simulink model "platform_screen_doors_multibody"  (R2024a)
settings: Solver=ode23t  StartTime=0.0  StopTime=12.5  MaxStep=0.00005  RelTol=1e-4  AbsTol=1e-3  EnableMultiTasking=on
undefined symbols (not defined in the file): X, Y, Z
libraries: fl_lib x27, nesl_utility x13, sm_lib x10, simulink x3, slpidlib x2
settings Model: Creator=USER  LastModifiedBy=Zeus
settings SolverCC: AutoScaleAbsTol=off  AlgebraicLoopSolver=TrustRegion  MaxZcPerStep=1
settings DataIOCC: LimitDataPoints=on  MaxDataPoints=10000  SaveFormat=Array
settings OptimizationCC: ReuseModelBlockBuffer=off  LifeSpan=inf
settings DebuggingCC: UnconnectedInputMsg=warning  UnconnectedOutputMsg=warning  UnconnectedLineMsg=warning  AllowSymbolicDim=off  SubsystemReferenceDiagnosticForUnitTest=warning  SFUnexpectedBacktrackingDiag=warning  SFNoUnconditionalDefaultTransitionDiag=warning  SFExecutionAtInitializationDiag=none  ArithmeticOperatorsInVariantConditions=warning
settings ModelReferenceCC: UpdateModelReferenceTargets=IfOutOfDate  EnableRefExpFcnMdlSchedulingChecks=on
settings SFSimCC: SimUseLocalCustomCode=off  CustomCodeUndefinedFunction=UseInterfaceOnly
settings RTWCC: RTWUseLocalCustomCode=off  GPUComputeCapability=3.5  DLArmComputeVersion=19.05
settings CodeAppCC: StateflowObjectComments=on
settings GRTTargetCC: TargetLangStandard=C89/C90 (ANSI)
settings ConfigComp: CovMetricSettings=dw  CovSaveCumulativeToWorkspaceVar=on  CovSaveSingleToWorkspaceVar=on  CovExternalEMLEnable=off  CovSFcnEnable=off
settings SimscapeCC: SimscapeLogType=all  SimscapeLogDataHistory=10000
settings ExplorerConfigSet: InternalSimMechanicsExplorerSettings=|
  | <ExplorerConfiguration>
  | 
  |   <canonicalview>default</canonicalview>
  | 
  |   <TilePanel>
  |     <TileInfo>
  |       <Tiles Columns="1" Count="1" Height="833" Rows="1" Width="1920">
  |         <Row Weight="1"/>
  |         <Column Weight="1"/>
  |         <Tile Height="1" Width="1" X="0" Y="0"/>
  |       </Tiles>
  |     </TileInfo>
  |     <SceneInfo>
  |       <SceneViewer>
  |         <IsThisViewStd>
  |           <IsStandardView>off</IsStandardView>
  |           <StandardViewName>Front</StandardViewName>
  |         </IsThisViewStd>
  |         <BGColor>
  |           <R>1</R>
  |           <G>1</G>
  |           <B>1</B>
  |           <A>1</A>
  |         </BGColor>
  |         <Camera>
  |           <DoPerspective>off</DoPerspective>
  |           <Position>
  |             <X>0.094040602001582485</X>
  |             <Y>-7.4533549176596825</Y>
  |             <Z>-0.037654221006226174</Z>
  |           </Position>
  |           <Center>
  |             <X>0.094040602001582485</X>
  |             <Y>0</Y>
  |             <Z>-0.037654221006226174</Z>
  |           </Center>
  |           <Up>
  |             <X>0</X>
  |             <Y>0</Y>
  |             <Z>1</Z>
  |           </Up>
  |           <XLim>1.1053593780096338</XLim>
  |           <YLim>1.1053593780096338</YLim>
  |           <ViewLimDist>0.01</ViewLimDist>
  |         </Camera>
  |       </SceneViewer>
  |     </SceneInfo>
  |   </TilePanel>
  | 
  |   <MechEditorPanel>
  |     <GfxPanelCameraMap/>
  |     <Cameras/>
  |     <VideoCreator>
  |       <IncludeTiles>All</IncludeTiles>
  |       <IncludeTime>on</IncludeTime>
  |       <IncludeWorldFrame>off</IncludeWorldFrame>
  |       <PlaybackSpeedRatio>1</PlaybackSpeedRatio>
  |       <FrameRate>30</FrameRate>
  |       <FrameSize>auto</FrameSize>
  |       <VideoFormat>MotionJPEGAVI</VideoFormat>
  |     </VideoCreator>
  |   </MechEditorPanel>
  | 
  |   <PlaybackSettings>
  |     <PlaybackSpeedFactor>1</PlaybackSpeedFactor>
  |   </PlaybackSettings>
  | 
  | </ExplorerConfiguration>

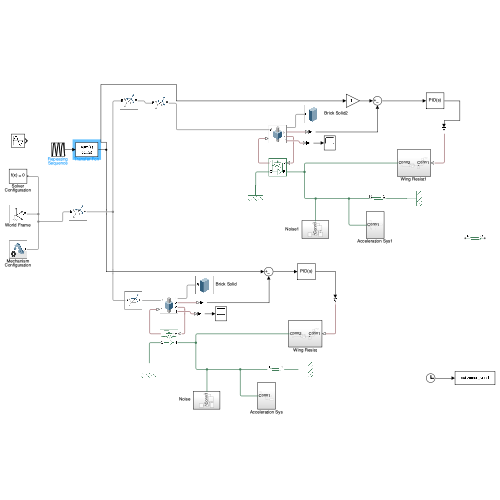
[thumbnail: Simulink's stored preview of the top-level diagram]
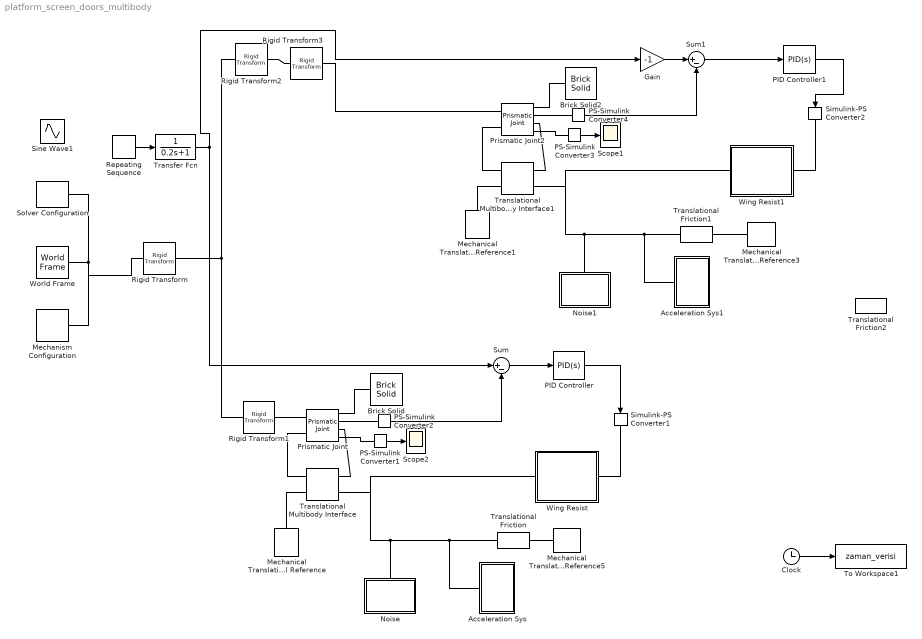
== system platform_screen_doors_multibody ==
  Acceleration Sys : Subsystem
  Acceleration Sys1 : Subsystem
  Brick Solid : sm_lib/Body Elements/Brick Solid  BrickDimensions=[1.9 0.05 0.8]  BrickDimensionsUnits=m  ExportEntireGeometry=off  InertiaType=PointMass  BasedOnType=Density  Density=1000  DensityUnits=kg/m^3  Mass=50  MassUnits=kg  CenterOfMass=[0 0 0]  CenterOfMassUnits=m  MomentsOfInertia=[1 1 1]  MomentsOfInertiaUnits=kg*m^2  ProductsOfInertia=[0 0 0]  ProductsOfInertiaUnits=kg*m^2  GraphicType=FromGeometry  MarkerShape=Sphere  MarkerSize=10  GraphicVisPropType=SimpleVisualProperties  GraphicDiffuseColor=[0.5 0.5 0.5]  GraphicOpacity=1.0  GraphicSpecularColor=[0.5 0.5 0.5 1.0]  GraphicAmbientColor=[0.15 0.15 0.15 1.0]  GraphicEmissiveColor=[0.0 0.0 0.0 1.0]  GraphicShininess=75  DoExposeReferenceFrame=on  SerializedFrames=<Frames/>
  Brick Solid2 : sm_lib/Body Elements/Brick Solid  BrickDimensions=[1.9 0.05 0.8]  BrickDimensionsUnits=m  ExportEntireGeometry=off  InertiaType=PointMass  BasedOnType=Density  Density=1000  DensityUnits=kg/m^3  Mass=50  MassUnits=kg  CenterOfMass=[0 0 0]  CenterOfMassUnits=m  MomentsOfInertia=[1 1 1]  MomentsOfInertiaUnits=kg*m^2  ProductsOfInertia=[0 0 0]  ProductsOfInertiaUnits=kg*m^2  GraphicType=FromGeometry  MarkerShape=Sphere  MarkerSize=10  GraphicVisPropType=SimpleVisualProperties  GraphicDiffuseColor=[0.5 0.5 0.5]  GraphicOpacity=1.0  GraphicSpecularColor=[0.5 0.5 0.5 1.0]  GraphicAmbientColor=[0.15 0.15 0.15 1.0]  GraphicEmissiveColor=[0.0 0.0 0.0 1.0]  GraphicShininess=75  DoExposeReferenceFrame=on  SerializedFrames=<Frames/>
  Clock : Clock
  Gain : Gain  Gain=-1
  Mechanical Translational Reference{,1,3,5} (4 alike) : fl_lib/Mechanical/Translational Elements/Mechanical Translational Reference
  Mechanism Configuration : sm_lib/Utilities/Mechanism Configuration  UniformGravity=Constant  GravityVector=[0 0 0]  GravityVectorUnits=m/s^2  LinearizationDelta=0.001  JointModeTransitionNonlinearIterations=2
  Noise : Subsystem
  Noise1 : Subsystem
  PID Controller : slpidlib/PID Controller  Controller=PID  Form=Parallel  TimeDomain=Continuous-time  UseExternalTs=off  SampleTime=-1  IntegratorMethod=Forward Euler  FilterMethod=Forward Euler  ControllerParametersSource=internal  P=10000  I=4000  UseKiTs=off  D=500  UseExternalDerivativeSource=off  N=100  UseFilter=on  TunerSelectOption=Transfer Function Based (PID Tuner App)  InitialConditionSource=internal  InitialConditionForIntegrator=0  InitialConditionForFilter=0  DifferentiatorICPrevScaledInput=0  ExternalReset=none  TrackingMode=off  Kt=1  LimitOutput=off  SatLimitsSource=internal  UpperSaturationLimit=inf  LowerSaturationLimit=-inf  LinearizeAsGain=on  AntiWindupMode=none  Kb=1  LimitIntegrator=off  UpperIntegratorSaturationLimit=inf  LowerIntegratorSaturationLimit=-inf  POutMin=[]  POutMax=[]  IOutMin=[]  IOutMax=[]  DOutMin=[]  DOutMax=[]  NOutMin=[]  NOutMax=[]  SumOutMin=[]  SumOutMax=[]  SaturationOutMin=[]  SaturationOutMax=[]  PParamMin=[]  PParamMax=[]  IParamMin=[]  IParamMax=[]  DParamMin=[]  DParamMax=[]  NParamMin=[]  NParamMax=[]  KbParamMin=[]  KbParamMax=[]  KtParamMin=[]  KtParamMax=[]  KbOutMin=[]  KbOutMax=[]  KtOutMin=[]  KtOutMax=[]  IntegratorOutMin=[]  IntegratorOutMax=[]  FilterOutMin=[]  FilterOutMax=[]  SumI1OutMin=[]  SumI1OutMax=[]  SumI2OutMin=[]  SumI2OutMax=[]  SumI3OutMin=[]  SumI3OutMax=[]  SumI4OutMin=[]  SumI4OutMax=[]  SumDOutMin=[]  SumDOutMax=[]  DifferentiatorOutMin=[]  DifferentiatorOutMax=[]  FilterDiffOutCoefMin=[]  FilterDiffOutCoefMax=[]  ReciprocalOutMin=[]  ReciprocalOutMax=[]  SumDenOutMin=[]  SumDenOutMax=[]  SumNumOutMin=[]  SumNumOutMax=[]  DivideOutMin=[]  DivideOutMax=[]  UdiffTsProdOutMin=[]  UdiffTsProdOutMax=[]  NTsProdOutMin=[]  NTsProdOutMax=[]  UintegralTsProdOutMin=[]  UintegralTsProdOutMax=[]  UngainTsProdOutMin=[]  UngainTsProdOutMax=[]  ClampingZeroOutDataTypeStr=Inherit: Inherit via back propagation  ClampingZeroOutMin=[]  ClampingZeroOutMax=[]  FilterDenConstantOutDataTypeStr=Inherit: Inherit via back propagation  FilterDenConstantOutMin=[]  FilterDenConstantOutMax=[]  PCopyOutDataTypeStr=Inherit: Inherit via back propagation  PCopyOutMin=[]  PCopyOutMax=[]  NCopyOutDataTypeStr=Inherit: Inherit via back propagation  NCopyOutMin=[]  NCopyOutMax=[]  IntegratorContinuousStateAttributes=''  IntegratorStateMustResolveToSignalObject=off  IntegratorRTWStateStorageClass=Auto  FilterContinuousStateAttributes=''  FilterStateMustResolveToSignalObject=off  FilterRTWStateStorageClass=Auto  ParallelPVariant=InternalParameters  IdealPVariant=Disabled  IVariant=InternalParameters  DVariant=InternalParameters  IntegratorVariant=Continuous  SatVariant=Disabled  AWVariant=Passthrough  PCopyVariant=Disabled  TRVariant=Disabled  FdbkBlocksVariant=Forward  IdealPFdbkVariant=Disabled  SatFdbkVariant=Disabled  DerivativeFilterVariant=ContFilter  NVariant=InternalParameters  NCopyVariant=Disabled  FilterICVariant=InternalICsFilter  IntegratorICVariant=InternalICs  ExternalResetVariant=Disabled  TRSumVariant=Passthrough  SumFdbkVariant=Disabled  SumVariant=Sum_PID  TsampFilterVariant=InternalTs  TsampNgainVariant=Passthrough  TsampIntegralVariant=Disabled_SignalSpec  ExternalSaturationOutDataTypeStr=Inherit: Same as second input  DerivativeSourceVariant=ErrorSignal
  PID Controller1 : slpidlib/PID Controller  Controller=PID  Form=Parallel  TimeDomain=Continuous-time  UseExternalTs=off  SampleTime=-1  IntegratorMethod=Forward Euler  FilterMethod=Forward Euler  ControllerParametersSource=internal  P=10000  I=4000  UseKiTs=off  D=500  UseExternalDerivativeSource=off  N=100  UseFilter=on  TunerSelectOption=Transfer Function Based (PID Tuner App)  InitialConditionSource=internal  InitialConditionForIntegrator=0  InitialConditionForFilter=0  DifferentiatorICPrevScaledInput=0  ExternalReset=none  TrackingMode=off  Kt=1  LimitOutput=off  SatLimitsSource=internal  UpperSaturationLimit=inf  LowerSaturationLimit=-inf  LinearizeAsGain=on  AntiWindupMode=none  Kb=1  LimitIntegrator=off  UpperIntegratorSaturationLimit=inf  LowerIntegratorSaturationLimit=-inf  POutMin=[]  POutMax=[]  IOutMin=[]  IOutMax=[]  DOutMin=[]  DOutMax=[]  NOutMin=[]  NOutMax=[]  SumOutMin=[]  SumOutMax=[]  SaturationOutMin=[]  SaturationOutMax=[]  PParamMin=[]  PParamMax=[]  IParamMin=[]  IParamMax=[]  DParamMin=[]  DParamMax=[]  NParamMin=[]  NParamMax=[]  KbParamMin=[]  KbParamMax=[]  KtParamMin=[]  KtParamMax=[]  KbOutMin=[]  KbOutMax=[]  KtOutMin=[]  KtOutMax=[]  IntegratorOutMin=[]  IntegratorOutMax=[]  FilterOutMin=[]  FilterOutMax=[]  SumI1OutMin=[]  SumI1OutMax=[]  SumI2OutMin=[]  SumI2OutMax=[]  SumI3OutMin=[]  SumI3OutMax=[]  SumI4OutMin=[]  SumI4OutMax=[]  SumDOutMin=[]  SumDOutMax=[]  DifferentiatorOutMin=[]  DifferentiatorOutMax=[]  FilterDiffOutCoefMin=[]  FilterDiffOutCoefMax=[]  ReciprocalOutMin=[]  ReciprocalOutMax=[]  SumDenOutMin=[]  SumDenOutMax=[]  SumNumOutMin=[]  SumNumOutMax=[]  DivideOutMin=[]  DivideOutMax=[]  UdiffTsProdOutMin=[]  UdiffTsProdOutMax=[]  NTsProdOutMin=[]  NTsProdOutMax=[]  UintegralTsProdOutMin=[]  UintegralTsProdOutMax=[]  UngainTsProdOutMin=[]  UngainTsProdOutMax=[]  ClampingZeroOutDataTypeStr=Inherit: Inherit via back propagation  ClampingZeroOutMin=[]  ClampingZeroOutMax=[]  FilterDenConstantOutDataTypeStr=Inherit: Inherit via back propagation  FilterDenConstantOutMin=[]  FilterDenConstantOutMax=[]  PCopyOutDataTypeStr=Inherit: Inherit via back propagation  PCopyOutMin=[]  PCopyOutMax=[]  NCopyOutDataTypeStr=Inherit: Inherit via back propagation  NCopyOutMin=[]  NCopyOutMax=[]  IntegratorContinuousStateAttributes=''  IntegratorStateMustResolveToSignalObject=off  IntegratorRTWStateStorageClass=Auto  FilterContinuousStateAttributes=''  FilterStateMustResolveToSignalObject=off  FilterRTWStateStorageClass=Auto  ParallelPVariant=InternalParameters  IdealPVariant=Disabled  IVariant=InternalParameters  DVariant=InternalParameters  IntegratorVariant=Continuous  SatVariant=Disabled  AWVariant=Passthrough  PCopyVariant=Disabled  TRVariant=Disabled  FdbkBlocksVariant=Forward  IdealPFdbkVariant=Disabled  SatFdbkVariant=Disabled  DerivativeFilterVariant=ContFilter  NVariant=InternalParameters  NCopyVariant=Disabled  FilterICVariant=InternalICsFilter  IntegratorICVariant=InternalICs  ExternalResetVariant=Disabled  TRSumVariant=Passthrough  SumFdbkVariant=Disabled  SumVariant=Sum_PID  TsampFilterVariant=InternalTs  TsampNgainVariant=Passthrough  TsampIntegralVariant=Disabled_SignalSpec  ExternalSaturationOutDataTypeStr=Inherit: Same as second input  DerivativeSourceVariant=ErrorSignal
  PS-Simulink Converter{1..4} (4 alike) : nesl_utility/PS-Simulink Converter  PhysicalDomain=network_engine_domain  SubClassName=ps_output  LeftPortType=input  RightPortType=output  PseudoPeriodic=off  Frequencies=[]  VectorFormat=inherit  Unit=inherit  AffineConversion=off
  Prismatic Joint : sm_lib/Joints/Prismatic Joint  JointMode=Normal  CompositeWrenchDir=FollowerOnBase  CompositeWrenchFrame=BaseFrame  SenseConstraintForce=off  SenseConstraintTorque=off  SenseTotalForce=off  SenseTotalTorque=off  PositionTargetSpecify=off  PositionTargetPriority=High  PositionTargetValue=0  PositionTargetValueUnits=m  VelocityTargetSpecify=off  VelocityTargetPriority=High  VelocityTargetValue=0  VelocityTargetValueUnits=m/s  EquilibriumPosition=0  EquilibriumPositionUnits=m  SpringStiffness=50  SpringStiffnessUnits=N/m  DampingCoefficient=10  DampingCoefficientUnits=N/(m/s)  LowerLimitSpecify=on  LowerLimitBound=0  LowerLimitBoundUnits=m  LowerLimitStiffness=1e6  LowerLimitStiffnessUnits=N/m  LowerLimitDamping=1e3  LowerLimitDampingUnits=N/(m/s)  LowerLimitTransitionRegionWidth=1e-4  LowerLimitTransitionRegionWidthUnits=m  UpperLimitSpecify=on  UpperLimitBound=0.8  UpperLimitBoundUnits=m  UpperLimitStiffness=1e6  UpperLimitStiffnessUnits=N/m  UpperLimitDamping=1e3  UpperLimitDampingUnits=N/(m/s)  UpperLimitTransitionRegionWidth=1e-4  UpperLimitTransitionRegionWidthUnits=m  TorqueActuationMode=InputTorque  MotionActuationMode=ComputedMotion  SensePosition=on  SenseVelocity=on  SenseAcceleration=off  SenseTorqueForce=on  SenseLowerLimitTorqueForce=off  SenseUpperLimitTorqueForce=off
  Prismatic Joint2 : sm_lib/Joints/Prismatic Joint  JointMode=Normal  CompositeWrenchDir=FollowerOnBase  CompositeWrenchFrame=BaseFrame  SenseConstraintForce=off  SenseConstraintTorque=off  SenseTotalForce=off  SenseTotalTorque=off  PositionTargetSpecify=off  PositionTargetPriority=High  PositionTargetValue=0  PositionTargetValueUnits=m  VelocityTargetSpecify=off  VelocityTargetPriority=High  VelocityTargetValue=0  VelocityTargetValueUnits=m/s  EquilibriumPosition=0  EquilibriumPositionUnits=m  SpringStiffness=50  SpringStiffnessUnits=N/m  DampingCoefficient=10  DampingCoefficientUnits=N/(m/s)  LowerLimitSpecify=on  LowerLimitBound=-0.8  LowerLimitBoundUnits=m  LowerLimitStiffness=1e6  LowerLimitStiffnessUnits=N/m  LowerLimitDamping=1e3  LowerLimitDampingUnits=N/(m/s)  LowerLimitTransitionRegionWidth=1e-4  LowerLimitTransitionRegionWidthUnits=m  UpperLimitSpecify=on  UpperLimitBound=0  UpperLimitBoundUnits=m  UpperLimitStiffness=1e6  UpperLimitStiffnessUnits=N/m  UpperLimitDamping=1e3  UpperLimitDampingUnits=N/(m/s)  UpperLimitTransitionRegionWidth=1e-4  UpperLimitTransitionRegionWidthUnits=m  TorqueActuationMode=InputTorque  MotionActuationMode=ComputedMotion  SensePosition=on  SenseVelocity=on  SenseAcceleration=off  SenseTorqueForce=on  SenseLowerLimitTorqueForce=off  SenseUpperLimitTorqueForce=off
  Repeating Sequence : simulink/Sources/Repeating Sequence  rep_seq_t="[0  1  4  5.5  8  11  12.5]"  rep_seq_y="[0  0  0.4  0.5  0.5  0.1  0]"
  Rigid Transform : sm_lib/Frames and Transforms/Rigid Transform  RotationMethod=StandardAxis  FollAlignAxisA=+X  BaseAlignAxisA=+Y  FollAlignAxisB=+Y  BaseAlignAxisB=+Z  RotationStandardAxis=+Y  RotationAngle=90  RotationAngleUnits=deg  RotationArbitraryAxis=[0 0 1]  RotationSequenceAxes=FollowerAxes  RotationSequence=XYX  RotationSequenceAngles=[0 0 0]  RotationSequenceAnglesUnits=deg  RotationMatrix=[1 0 0;0 1 0;0 0 1]  Quaternion=[1 0 0 0]  TranslationMethod=None  TranslationCartesianOffset=[0 0 0]  TranslationCartesianOffsetUnits=m  TranslationStandardAxis=+Z  TranslationStandardOffset=0  TranslationStandardOffsetUnits=m  TranslationROffset=0  TranslationROffsetUnits=m  TranslationThetaOffset=0  TranslationThetaOffsetUnits=deg  TranslationZOffset=0  TranslationZOffsetUnits=m
  Rigid Transform1 : sm_lib/Frames and Transforms/Rigid Transform  RotationMethod=None  FollAlignAxisA=+X  BaseAlignAxisA=+Y  FollAlignAxisB=+Y  BaseAlignAxisB=+Z  RotationStandardAxis=+Y  RotationAngle=0  RotationAngleUnits=deg  RotationArbitraryAxis=[0 0 1]  RotationSequenceAxes=FollowerAxes  RotationSequence=XYX  RotationSequenceAngles=[0 0 0]  RotationSequenceAnglesUnits=deg  RotationMatrix=[1 0 0;0 1 0;0 0 1]  Quaternion=[1 0 0 0]  TranslationMethod=StandardAxis  TranslationCartesianOffset=[0 0 0]  TranslationCartesianOffsetUnits=m  TranslationStandardAxis=+Z  TranslationStandardOffset=+0.2  TranslationStandardOffsetUnits=m  TranslationROffset=0  TranslationROffsetUnits=m  TranslationThetaOffset=0  TranslationThetaOffsetUnits=deg  TranslationZOffset=0  TranslationZOffsetUnits=m
  Rigid Transform2 : sm_lib/Frames and Transforms/Rigid Transform  RotationMethod=None  FollAlignAxisA=+X  BaseAlignAxisA=+Y  FollAlignAxisB=+Y  BaseAlignAxisB=+Z  RotationStandardAxis=+Y  RotationAngle=0  RotationAngleUnits=deg  RotationArbitraryAxis=[0 0 1]  RotationSequenceAxes=FollowerAxes  RotationSequence=XYX  RotationSequenceAngles=[0 0 0]  RotationSequenceAnglesUnits=deg  RotationMatrix=[1 0 0;0 1 0;0 0 1]  Quaternion=[1 0 0 0]  TranslationMethod=StandardAxis  TranslationCartesianOffset=[0 0 0]  TranslationCartesianOffsetUnits=m  TranslationStandardAxis=+Z  TranslationStandardOffset=-0.4  TranslationStandardOffsetUnits=m  TranslationROffset=0  TranslationROffsetUnits=m  TranslationThetaOffset=0  TranslationThetaOffsetUnits=deg  TranslationZOffset=0  TranslationZOffsetUnits=m
  Rigid Transform3 : sm_lib/Frames and Transforms/Rigid Transform  RotationMethod=None  FollAlignAxisA=+X  BaseAlignAxisA=+Y  FollAlignAxisB=+Y  BaseAlignAxisB=+Z  RotationStandardAxis=+Y  RotationAngle=0  RotationAngleUnits=deg  RotationArbitraryAxis=[0 0 1]  RotationSequenceAxes=FollowerAxes  RotationSequence=XYX  RotationSequenceAngles=[0 0 0]  RotationSequenceAnglesUnits=deg  RotationMatrix=[1 0 0;0 1 0;0 0 1]  Quaternion=[1 0 0 0]  TranslationMethod=StandardAxis  TranslationCartesianOffset=[0 0 0]  TranslationCartesianOffsetUnits=m  TranslationStandardAxis=+Z  TranslationStandardOffset=-0.2  TranslationStandardOffsetUnits=m  TranslationROffset=0  TranslationROffsetUnits=m  TranslationThetaOffset=0  TranslationThetaOffsetUnits=deg  TranslationZOffset=0  TranslationZOffsetUnits=m
  Scope1 : Scope
  Scope2 : Scope
  Simulink-PS Converter1 : nesl_utility/Simulink-PS Converter  PhysicalDomain=network_engine_domain  SubClassName=ps_input  LeftPortType=input  RightPortType=output  PseudoPeriodic=off  Frequencies=[]  NoiseDistribution=none  NoiseParameters=[]  Unit=1  AffineConversion=off  FilteringAndDerivatives=provide  SimscapeFilterOrder=1  InputFilterTimeConstant=0.001  UdotUserProvided=0
  Simulink-PS Converter2 : nesl_utility/Simulink-PS Converter  PhysicalDomain=network_engine_domain  SubClassName=ps_input  LeftPortType=input  RightPortType=output  PseudoPeriodic=off  Frequencies=[]  NoiseDistribution=none  NoiseParameters=[]  Unit=1  AffineConversion=off  FilteringAndDerivatives=provide  SimscapeFilterOrder=1  InputFilterTimeConstant=0.001  UdotUserProvided=0
  Sine Wave1 : Sin  Amplitude=0.3  Bias=0.3  Phase=-1.57  SampleTime=0
  Solver Configuration : nesl_utility/Solver Configuration  PhysicalDomain=network_engine_domain  SubClassName=solver  LeftPortType=input  RightPortType=generic  Tones=[]  Harmonics=[]  SimulateNoise=off  Profile=off  UseLocalSampling=off  EnableSwitchedLinearOptims=on  FrequencyDomain=off  UseCCode=off  RelTol=0.001  AbsTol=1e-06  MinStep=1e-09  ToWorkspace=off  RevertToSquareIcSolve=off  NumHomotopyIterations=100  PhasorMode=off  PhasorModeNumHarmonics=1  ConsistencySolver=NEWTON_XTOL_AFTER_FTOL  IndexReductionMethod=DerivativeReplacement  DoDC=off  ResidualTolerance=1e-09  ConsistencyTolSource=GLOBAL  ConsistencyAbsTol=0.001  ConsistencyRelTol=0.001  ConsistencyTolFactor=0.001  UseLocalSolver=off  LocalSolverChoice=NE_BACKWARD_EULER_ADVANCER  ResolveIndetEquations=on  FunctionEvalNumThread=1  LocalSolverSampleTime=0.001  DoFixedCost=off  MaxNonlinIter=3  MaxModeIter=2  ComputeImpulses=off  ImpulseIterations=2  LinearAlgebra=Sparse  LinearAlgebraNumThread=0  EquationFormulation=NE_TIME_EF  DelaysMemoryBudget=1024  AutomaticFiltering=on  FilteringTimeConstant=0.001  PartitionStorageMethod=AS_NEEDED  PartitionMemoryBudget=1024  PartitionMethod=FAST  MultibodyUseLocalSolver=off  MultibodyLocalSolverChoice=ODE1  MultibodyLocalSolverSampleTime=0.001
  Sum : Sum  Inputs=|+-
  Sum1 : Sum  Inputs=|+-
  To Workspace1 : ToWorkspace  VariableName=zaman_verisi  SampleTime=-1
  Transfer Fcn : TransferFcn  Denominator=[0.2 1]
  Translational Friction : fl_lib/Mechanical/Translational Elements/Translational Friction  brkwy_frc=200 N  brkwy_vel=0.05 m/s  Col_frc=150 N  visc_coef=0 N*s/m  v_specify=off  v_priority=None  v=0 m/s  v_nominal_specify=off  v_nominal_value=1  v_nominal_unit=m/s  f_specify=off  f_priority=None  f=0 N  f_nominal_specify=off  f_nominal_value=1  f_nominal_unit=N
      settings: InternalSimscapePortConfiguration="{\"Bottom\":[],\"Left\":[{\"id\":\"R\",\"label\":\"R\",\"type\":\"foundation.mechanical.translational.translational\"}],\"Right\":[{\"id\":\"C\",\"label\":\"C\",\"type\":\"foundation.mechanical.translational.translational\"}],\"Top\":[]}"
  Translational Friction1 : fl_lib/Mechanical/Translational Elements/Translational Friction  brkwy_frc=200 N  brkwy_vel=0.05 m/s  Col_frc=150 N  visc_coef=0 N*s/m  v_specify=off  v_priority=None  v=0 m/s  v_nominal_specify=off  v_nominal_value=1  v_nominal_unit=m/s  f_specify=off  f_priority=None  f=0 N  f_nominal_specify=off  f_nominal_value=1  f_nominal_unit=N
      settings: InternalSimscapePortConfiguration="{\"Bottom\":[],\"Left\":[{\"id\":\"R\",\"label\":\"R\",\"type\":\"foundation.mechanical.translational.translational\"}],\"Right\":[{\"id\":\"C\",\"label\":\"C\",\"type\":\"foundation.mechanical.translational.translational\"}],\"Top\":[]}"
  Translational Friction2 : fl_lib/Mechanical/Translational Elements/Translational Friction  brkwy_frc=100 N  brkwy_vel=0.05 m/s  Col_frc=100 N  visc_coef=0 N*s/m  v_specify=off  v_priority=None  v=0 m/s  v_nominal_specify=off  v_nominal_value=1  v_nominal_unit=m/s  f_specify=off  f_priority=None  f=0 N  f_nominal_specify=off  f_nominal_value=1  f_nominal_unit=N
      settings: InternalSimscapePortConfiguration="{\"Bottom\":[],\"Left\":[{\"id\":\"R\",\"label\":\"R\",\"type\":\"foundation.mechanical.translational.translational\"}],\"Right\":[{\"id\":\"C\",\"label\":\"C\",\"type\":\"foundation.mechanical.translational.translational\"}],\"Top\":[]}"
  Translational Multibody Interface : fl_lib/Mechanical/Multibody Interfaces/Translational Multibody Interface
  Translational Multibody Interface1 : fl_lib/Mechanical/Multibody Interfaces/Translational Multibody Interface
  Wing Resist : Subsystem
  Wing Resist1 : Subsystem
  World Frame : sm_lib/Frames and Transforms/World Frame
  wires:
  Repeating Sequence/1 -> Transfer Fcn/1
  PS-Simulink Converter1/1 -> Scope2/1
  PS-Simulink Converter2/1 -> Sum/2
  Sum/1 -> PID Controller/1
  PID Controller/1 -> Simulink-PS Converter1/1
  Clock/1 -> To Workspace1/1
  PS-Simulink Converter3/1 -> Scope1/1
  PS-Simulink Converter4/1 -> Sum1/2
  PID Controller1/1 -> Simulink-PS Converter2/1
  Sum1/1 -> PID Controller1/1
  Gain/1 -> Sum1/1
  Transfer Fcn/1 -> Sum/1, Gain/1
  connections:
  World Frame/RConn1 -- Rigid Transform/LConn1 -- Mechanism Configuration/RConn1 -- Solver Configuration/RConn1
  Brick Solid/RConn1 -- Prismatic Joint/RConn1
  Prismatic Joint/RConn4 -- PS-Simulink Converter1/LConn1
  Prismatic Joint/LConn1 -- Rigid Transform1/RConn1
  Rigid Transform1/LConn1 -- Rigid Transform2/LConn1 -- Rigid Transform/RConn1
  Rigid Transform2/RConn1 -- Rigid Transform3/LConn1
  Rigid Transform3/RConn1 -- Prismatic Joint2/LConn1
  Translational Multibody Interface/RConn1 -- Prismatic Joint/RConn3
  Translational Multibody Interface/LConn1 -- Prismatic Joint/LConn2
  Translational Multibody Interface/LConn2 -- Mechanical Translational Reference/LConn1
  PS-Simulink Converter2/LConn1 -- Prismatic Joint/RConn2
  Mechanical Translational Reference5/LConn1 -- Translational Friction/RConn1
  Noise/LConn1 -- Wing Resist/LConn1 -- Translational Multibody Interface/RConn2 -- Acceleration Sys/LConn1 -- Translational Friction/LConn1
  Wing Resist/RConn1 -- Simulink-PS Converter1/RConn1
  Wing Resist1/LConn1 -- Translational Multibody Interface1/RConn2 -- Noise1/LConn1 -- Translational Friction1/LConn1 -- Acceleration Sys1/LConn1
  Translational Friction1/RConn1 -- Mechanical Translational Reference3/LConn1
  Prismatic Joint2/RConn4 -- PS-Simulink Converter3/LConn1
  Brick Solid2/RConn1 -- Prismatic Joint2/RConn1
  Translational Multibody Interface1/RConn1 -- Prismatic Joint2/RConn3
  PS-Simulink Converter4/LConn1 -- Prismatic Joint2/RConn2
  Wing Resist1/RConn1 -- Simulink-PS Converter2/RConn1
  Prismatic Joint2/LConn2 -- Translational Multibody Interface1/LConn1
  Mechanical Translational Reference1/LConn1 -- Translational Multibody Interface1/LConn2

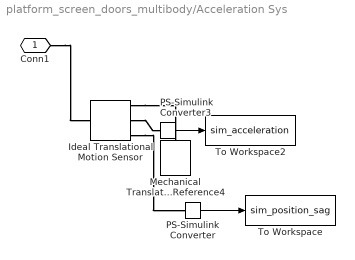
== system platform_screen_doors_multibody/Acceleration Sys ==
  Ideal Translational Motion Sensor : fl_lib/Mechanical/Mechanical Sensors/Ideal Translational Motion Sensor  reference=foundation.enum.MeasurementReference.difference  acceleration_port=true  velocity_port=false  position_port=true  offset=0 m
      settings: InternalSimscapePortConfiguration="{\"Bottom\":[],\"Left\":[{\"id\":\"R\",\"label\":\"R\",\"type\":\"foundation.mechanical.translational.translational\"}],\"Right\":[{\"id\":\"C\",\"label\":\"C\",\"type\":\"foundation.mechanical.translational.translational\"},{\"id\":\"A\",\"label\":\"A\",\"type\":\"output\"},{\"id\":\"P\",\"label\":\"P\",\"type\":\"output\"}],\"Top\":[]}"
  Mechanical Translational Reference4 : fl_lib/Mechanical/Translational Elements/Mechanical Translational Reference
  PS-Simulink Converter : nesl_utility/PS-Simulink Converter  PhysicalDomain=network_engine_domain  SubClassName=ps_output  LeftPortType=input  RightPortType=output  PseudoPeriodic=off  Frequencies=[]  VectorFormat=inherit  Unit=inherit  AffineConversion=off
  PS-Simulink Converter3 : nesl_utility/PS-Simulink Converter  PhysicalDomain=network_engine_domain  SubClassName=ps_output  LeftPortType=input  RightPortType=output  PseudoPeriodic=off  Frequencies=[]  VectorFormat=inherit  Unit=inherit  AffineConversion=off
  To Workspace : ToWorkspace  VariableName=sim_position_sag  SaveFormat=Timeseries  SampleTime=-1
  To Workspace2 : ToWorkspace  VariableName=sim_acceleration  SampleTime=-1
  Conn1 : PMIOPort  Side=Left
  wires:
  PS-Simulink Converter3/1 -> To Workspace2/1
  PS-Simulink Converter/1 -> To Workspace/1
  connections:
  Ideal Translational Motion Sensor/RConn2 -- PS-Simulink Converter3/LConn1
  Conn1/RConn1 -- Ideal Translational Motion Sensor/LConn1
  Ideal Translational Motion Sensor/RConn1 -- Mechanical Translational Reference4/LConn1
  Ideal Translational Motion Sensor/RConn3 -- PS-Simulink Converter/LConn1

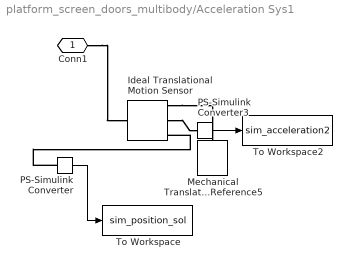
== system platform_screen_doors_multibody/Acceleration Sys1 ==
  Ideal Translational Motion Sensor : fl_lib/Mechanical/Mechanical Sensors/Ideal Translational Motion Sensor  reference=foundation.enum.MeasurementReference.difference  acceleration_port=true  velocity_port=false  position_port=true  offset=0 m
      settings: InternalSimscapePortConfiguration="{\"Bottom\":[],\"Left\":[{\"id\":\"R\",\"label\":\"R\",\"type\":\"foundation.mechanical.translational.translational\"}],\"Right\":[{\"id\":\"C\",\"label\":\"C\",\"type\":\"foundation.mechanical.translational.translational\"},{\"id\":\"A\",\"label\":\"A\",\"type\":\"output\"},{\"id\":\"P\",\"label\":\"P\",\"type\":\"output\"}],\"Top\":[]}"
  Mechanical Translational Reference5 : fl_lib/Mechanical/Translational Elements/Mechanical Translational Reference
  PS-Simulink Converter : nesl_utility/PS-Simulink Converter  PhysicalDomain=network_engine_domain  SubClassName=ps_output  LeftPortType=input  RightPortType=output  PseudoPeriodic=off  Frequencies=[]  VectorFormat=inherit  Unit=inherit  AffineConversion=off
  PS-Simulink Converter3 : nesl_utility/PS-Simulink Converter  PhysicalDomain=network_engine_domain  SubClassName=ps_output  LeftPortType=input  RightPortType=output  PseudoPeriodic=off  Frequencies=[]  VectorFormat=inherit  Unit=inherit  AffineConversion=off
  To Workspace : ToWorkspace  VariableName=sim_position_sol  SaveFormat=Timeseries  SampleTime=-1
  To Workspace2 : ToWorkspace  VariableName=sim_acceleration2  SampleTime=-1
  Conn1 : PMIOPort  Side=Left
  wires:
  PS-Simulink Converter3/1 -> To Workspace2/1
  PS-Simulink Converter/1 -> To Workspace/1
  connections:
  Ideal Translational Motion Sensor/RConn2 -- PS-Simulink Converter3/LConn1
  Conn1/RConn1 -- Ideal Translational Motion Sensor/LConn1
  Ideal Translational Motion Sensor/RConn1 -- Mechanical Translational Reference5/LConn1
  PS-Simulink Converter/LConn1 -- Ideal Translational Motion Sensor/RConn3

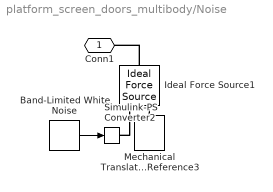
== system platform_screen_doors_multibody/Noise ==
  Band-Limited White Noise : simulink/Sources/Band-Limited White Noise  Cov=0.2  Ts=0.01  seed=[23341]
  Ideal Force Source1 : fl_lib/Mechanical/Mechanical Sources/Ideal Force Source
  Mechanical Translational Reference3 : fl_lib/Mechanical/Translational Elements/Mechanical Translational Reference
  Simulink-PS Converter2 : nesl_utility/Simulink-PS Converter  PhysicalDomain=network_engine_domain  SubClassName=ps_input  LeftPortType=input  RightPortType=output  PseudoPeriodic=off  Frequencies=[]  NoiseDistribution=none  NoiseParameters=[]  Unit=1  AffineConversion=off  FilteringAndDerivatives=provide  SimscapeFilterOrder=1  InputFilterTimeConstant=0.001  UdotUserProvided=0
  Conn1 : PMIOPort  Side=Left
  wires:
  Band-Limited White Noise/1 -> Simulink-PS Converter2/1
  connections:
  Ideal Force Source1/LConn1 -- Conn1/RConn1
  Mechanical Translational Reference3/LConn1 -- Ideal Force Source1/RConn2
  Ideal Force Source1/RConn1 -- Simulink-PS Converter2/RConn1

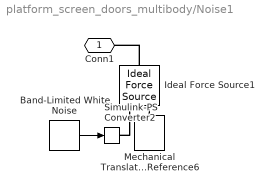
== system platform_screen_doors_multibody/Noise1 ==
  Band-Limited White Noise : simulink/Sources/Band-Limited White Noise  Cov=0.2  Ts=0.01  seed=[23341]
  Ideal Force Source1 : fl_lib/Mechanical/Mechanical Sources/Ideal Force Source
  Mechanical Translational Reference6 : fl_lib/Mechanical/Translational Elements/Mechanical Translational Reference
  Simulink-PS Converter2 : nesl_utility/Simulink-PS Converter  PhysicalDomain=network_engine_domain  SubClassName=ps_input  LeftPortType=input  RightPortType=output  PseudoPeriodic=off  Frequencies=[]  NoiseDistribution=none  NoiseParameters=[]  Unit=1  AffineConversion=off  FilteringAndDerivatives=filter  SimscapeFilterOrder=1  InputFilterTimeConstant=0.001  UdotUserProvided=0
  Conn1 : PMIOPort  Side=Left
  wires:
  Band-Limited White Noise/1 -> Simulink-PS Converter2/1
  connections:
  Ideal Force Source1/LConn1 -- Conn1/RConn1
  Mechanical Translational Reference6/LConn1 -- Ideal Force Source1/RConn2
  Ideal Force Source1/RConn1 -- Simulink-PS Converter2/RConn1

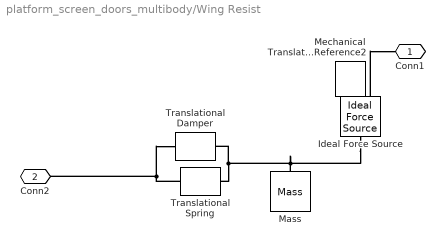
== system platform_screen_doors_multibody/Wing Resist ==
  Ideal Force Source : fl_lib/Mechanical/Mechanical Sources/Ideal Force Source
  Mass : fl_lib/Mechanical/Translational Elements/Mass  mass=10 kg  num_ports=foundation.enum.numPorts2.one  v_specify=off  v_priority=High  v=0 m/s  v_nominal_specify=off  v_nominal_value=1  v_nominal_unit=m/s  f_specify=off  f_priority=None  f=0 N  f_nominal_specify=off  f_nominal_value=1  f_nominal_unit=N
  Mechanical Translational Reference2 : fl_lib/Mechanical/Translational Elements/Mechanical Translational Reference
  Translational Damper : fl_lib/Mechanical/Translational Elements/Translational Damper  D=170 N*s/m  v_specify=off  v_priority=None  v=0 m/s  v_nominal_specify=off  v_nominal_value=1  v_nominal_unit=m/s  f_specify=off  f_priority=None  f=0 N  f_nominal_specify=off  f_nominal_value=1  f_nominal_unit=N
  Translational Spring : fl_lib/Mechanical/Translational Elements/Translational Spring  spr_rate=15000 N/m  v_specify=off  v_priority=None  v=0 m/s  v_nominal_specify=off  v_nominal_value=1  v_nominal_unit=m/s  f_specify=off  f_priority=None  f=0 N  f_nominal_specify=off  f_nominal_value=1  f_nominal_unit=N  x_specify=off  x_priority=High  x=0 m  x_nominal_specify=off  x_nominal_value=1  x_nominal_unit=m
  Conn1 : PMIOPort  Side=Right
  Conn2 : PMIOPort  Port=2  Side=Left
  connections:
  Translational Spring/RConn1 -- Translational Damper/RConn1 -- Conn2/RConn1
  Ideal Force Source/RConn1 -- Conn1/RConn1
  Mass/LConn1 -- Ideal Force Source/LConn1 -- Translational Damper/LConn1 -- Translational Spring/LConn1
  Ideal Force Source/RConn2 -- Mechanical Translational Reference2/LConn1

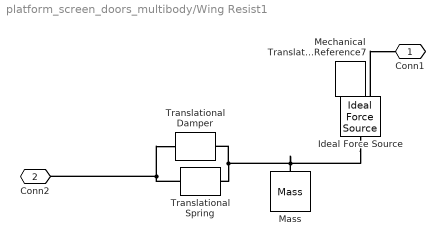
== system platform_screen_doors_multibody/Wing Resist1 ==
  Ideal Force Source : fl_lib/Mechanical/Mechanical Sources/Ideal Force Source
  Mass : fl_lib/Mechanical/Translational Elements/Mass  mass=10 kg  num_ports=foundation.enum.numPorts2.one  v_specify=off  v_priority=High  v=0 m/s  v_nominal_specify=off  v_nominal_value=1  v_nominal_unit=m/s  f_specify=off  f_priority=None  f=0 N  f_nominal_specify=off  f_nominal_value=1  f_nominal_unit=N
  Mechanical Translational Reference7 : fl_lib/Mechanical/Translational Elements/Mechanical Translational Reference
  Translational Damper : fl_lib/Mechanical/Translational Elements/Translational Damper  D=170 N*s/m  v_specify=off  v_priority=None  v=0 m/s  v_nominal_specify=off  v_nominal_value=1  v_nominal_unit=m/s  f_specify=off  f_priority=None  f=0 N  f_nominal_specify=off  f_nominal_value=1  f_nominal_unit=N
  Translational Spring : fl_lib/Mechanical/Translational Elements/Translational Spring  spr_rate=15000 N/m  v_specify=off  v_priority=None  v=0 m/s  v_nominal_specify=off  v_nominal_value=1  v_nominal_unit=m/s  f_specify=off  f_priority=None  f=0 N  f_nominal_specify=off  f_nominal_value=1  f_nominal_unit=N  x_specify=off  x_priority=High  x=0 m  x_nominal_specify=off  x_nominal_value=1  x_nominal_unit=m
  Conn1 : PMIOPort  Side=Right
  Conn2 : PMIOPort  Port=2  Side=Left
  connections:
  Translational Spring/RConn1 -- Conn2/RConn1 -- Translational Damper/RConn1
  Ideal Force Source/RConn1 -- Conn1/RConn1
  Mass/LConn1 -- Translational Damper/LConn1 -- Translational Spring/LConn1 -- Ideal Force Source/LConn1
  Ideal Force Source/RConn2 -- Mechanical Translational Reference7/LConn1
